simulink model "ToyLibRef"  (R2023b)
settings: Solver=VariableStepAuto  StartTime=0.0  StopTime=10.0  RelTol=1e-3
libraries: ToyLib x4
settings Model: Creator=na  LastModifiedBy=na

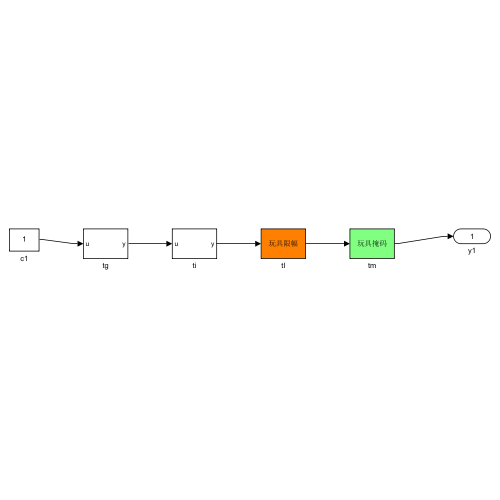
[thumbnail: Simulink's stored preview of the top-level diagram]
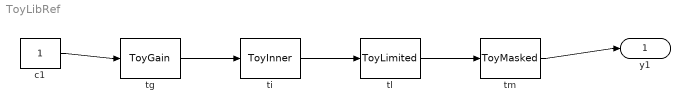
== system ToyLibRef ==
  c1 : Constant
  tg : ToyLib/ToyGain  SystemSampleTime=-1  VariantActivationTime=update diagram  AllowFlexibleInterface=on  Latency=0  AutoFrameSizeCalculation=off
  ti : ToyLib/ToyInner  SystemSampleTime=-1  VariantActivationTime=update diagram  AllowFlexibleInterface=on  Latency=0  AutoFrameSizeCalculation=off
  tl : ToyLib/ToyLimited  UpperLimit=1
  tm : ToyLib/ToyMasked  Kp=5
  y1 : Outport
  wires:
  c1/1 -> tg/1
  tg/1 -> ti/1
  ti/1 -> tl/1
  tl/1 -> tm/1
  tm/1 -> y1/1
